simulink model "MOBATSim"  (R2020b)
settings: Solver=FixedStepAuto  StartTime=0.0  StopTime=Sim_t  FixedStep=0.01  MinStep=0.01  RelTol=1e-2
values from neighbouring files (symbols this model uses):
  Vehicles = evalin('base','Vehicles')    [I2V.m]    (also in VehicleSensors.m)
undefined symbols (not defined in the file or in its folder): Sim_Ts
libraries: simulink x50, robotalgslib x10, drivingvehiclecontroller x10, mpcadaslib x10, pid_lib x10
(part 3 of 7)

== system MOBATSim/Vehicle Model 7/Vehicle Model ==
  Longitudinal Speed : Inport
  Steering Angle : Inport  Port=2
  Delay : Delay  DelayLength=1  SampleTime=Sim_Ts
  Kinematic Bicycle Model : Subsystem
  Selector3 : Selector  InputPortWidth=3  IndexOptions=Index vector (dialog)  Indices=[1]  OutputSizes=1
  Selector4 : Selector  InputPortWidth=3  IndexOptions=Index vector (dialog)  Indices=[2]  OutputSizes=1
  Sqrt : Sqrt  SaturateOnIntegerOverflow=on
  Square : Math  Operator=square  SaturateOnIntegerOverflow=on
  Square1 : Math  Operator=square  SaturateOnIntegerOverflow=on
  Sum1 : Sum  Inputs=|++
  Zero-Order Hold1 : ZeroOrderHold  SampleTime=Sim_Ts
  Zero-Order Hold2 : ZeroOrderHold  SampleTime=Sim_Ts
  Pose : Outport
  Speed : Outport  Port=2
  wires:
  Delay/1 -> Speed/1
  Kinematic Bicycle Model/1(state) -> Zero-Order Hold1/1
  Selector4/1 -> Square1/1
  Longitudinal Speed/1 -> Kinematic Bicycle Model/1(v)
  Steering Angle/1 -> Kinematic Bicycle Model/2(Steering Angle)
  Sum1/1 -> Sqrt/1
  Sqrt/1 -> Delay/1
  Square/1 -> Sum1/1
  Square1/1 -> Sum1/2
  Selector3/1 -> Square/1
  Kinematic Bicycle Model/2(stateDot) -> Zero-Order Hold2/1
  Zero-Order Hold1/1 -> Pose/1
  Zero-Order Hold2/1 -> Selector4/1, Selector3/1

== system MOBATSim/Vehicle Model 7/Vehicle Status Check and Acceleration to Speed ==
  note: Longitudinal
  Reference Acceleration : Inport
  Reference Steering Angle : Inport  Port=2
  Acceleration to Speed : Integrator  LimitOutput=on  LowerSaturationLimit=0
  MATLAB System : MATLABSystem  System=VehicleStopStatusCheck  Vehicle_id=Vehicle_id  SimulateUsing=Interpreted execution
      mask Type: VehicleStopStatusCheck
      mask Display:
      | disp('VehicleStopStatusCheck');
      | port_label('input',1,'Acc');
      | port_label('input',2,'Steering');
      | port_label('output',1,'Acc');
      | port_label('output',2,'Stop');
      | port_label('output',3,'Steering');
  Product : Product
  Signal Specification : SignalSpecification  Dimensions=1
  Stop Check : simulink/Logic and Bit Operations/Compare To Constant  relop=~=  const=1  OutDataTypeStr=uint8
  Zero-Order Hold : ZeroOrderHold  SampleTime=Sim_Ts
  Speed Cmd : Outport
  Steering Angle Cmd : Outport  Port=2
  wires:
  Acceleration to Speed/1 -> Signal Specification/1
  Stop Check/1 -> Product/2
  MATLAB System/3 -> Steering Angle Cmd/1
  Signal Specification/1 -> Zero-Order Hold/1
  Reference Acceleration/1 -> MATLAB System/1
  Zero-Order Hold/1 -> Product/1
  Product/1 -> Speed Cmd/1
  MATLAB System/1 -> Acceleration to Speed/1
  Reference Steering Angle/1 -> MATLAB System/2
  MATLAB System/2 -> Stop Check/1

== system MOBATSim/Vehicle Model 8/Longitudinal and Lateral Controllers ==
  Speed Reference : Inport
  Inter Vehicular Distance : Inport  Port=2
  Lead Speed : Inport  Port=3
  drivingMode : Inport  Port=4
  Dist2Stop : Inport  Port=5
  laneChange : Inport  Port=6
  Actual Pose : Inport  Port=7
  Actual Speed : Inport  Port=8
  Lateral Motion Control : Subsystem  Variant=on  VariantControlMode=label  LabelModeActiveChoice=STANLEY  mask{modeLateral=STANLEY}
      mask prompts: modeLateral "Lateral Control Mode:"
      mask TypeOptions modeLateral: PURE_PURSUIT | STANLEY
      mask Callback modeLateral: set_param(gcb,'OverrideUsingVariant',get_param(gcb,'modeLateral'));
  Longitudinal Speed Control : Subsystem
  Longitudinal Acceleration Cmd : Outport
  Reference Steering Angle : Outport  Port=2
  wires:
  laneChange/1 -> Lateral Motion Control/3(changeLane)
  Lateral Motion Control/1(SteerCmd) -> Reference Steering Angle/1
  Actual Speed/1 -> Lateral Motion Control/1(speed), Longitudinal Speed Control/6(Actual Speed)
  drivingMode/1 -> Longitudinal Speed Control/4(Driving Mode)
  Longitudinal Speed Control/1(Longitduinal Acceleration Command) -> Longitudinal Acceleration Cmd/1
  Dist2Stop/1 -> Longitudinal Speed Control/5(Dist2Stop)
  Inter Vehicular Distance/1 -> Longitudinal Speed Control/2(Inter Vehicular Distance)
  Lead Speed/1 -> Longitudinal Speed Control/3(Lead Speed)
  Speed Reference/1 -> Longitudinal Speed Control/1(Speed Reference)
  Actual Pose/1 -> Lateral Motion Control/2(pose)

== system MOBATSim/Vehicle Model 8/Path Planner ==
  note: 1) Add Subsystem or Model blocks as valid variant choices.
      | 2) You cannot connect blocks at this level. At simulation, connectivity is automatically
      | determined, based on the active variant and port name matching.
  CommunicationIDs : Inport
  Astar : Subsystem  VariantControl=Astar
  ShortestPathFinder : Subsystem  VariantControl=ShortestPathFinder
  waypointReached : Outport

== system MOBATSim/Vehicle Model 8/Transform to MOBATSim Coordinates ==
  Pose : Inport
  Constant : Constant  Value=0
  Constant1 : Constant
  Constant2 : Constant  Value=0
  Constant3 : Constant  Value=0
  Constant4 : Constant  Value=pi/2
  Gain : Gain  Gain=-1
  Matrix Concatenate : Concatenate  NumInputs=4  ConcatenateDimension=2
  Matrix Concatenate1 : Concatenate  NumInputs=3  ConcatenateDimension=2
  Selector1 : Selector  InputPortWidth=3  IndexOptions=Index vector (dialog)  Indices=[3]  OutputSizes=1
  Selector3 : Selector  InputPortWidth=3  IndexOptions=Index vector (dialog)  Indices=[1]  OutputSizes=1
  Selector4 : Selector  InputPortWidth=3  IndexOptions=Index vector (dialog)  Indices=[2]  OutputSizes=1
  Sum : Sum  Inputs=|++
  Position : Outport
  Orientation : Outport  Port=2
  wires:
  Sum/1 -> Matrix Concatenate/4
  Constant2/1 -> Matrix Concatenate/1
  Constant3/1 -> Matrix Concatenate1/2
  Gain/1 -> Matrix Concatenate1/3
  Constant4/1 -> Sum/2
  Constant1/1 -> Matrix Concatenate/2
  Selector1/1 -> Sum/1
  Constant/1 -> Matrix Concatenate/3
  Matrix Concatenate/1 -> Orientation/1
  Matrix Concatenate1/1 -> Position/1
  Selector4/1 -> Gain/1
  Selector3/1 -> Matrix Concatenate1/1
  Pose/1 -> Selector1/1, Selector4/1, Selector3/1

== system MOBATSim/Vehicle Model 8/Vehicle Model ==
  Longitudinal Speed : Inport
  Steering Angle : Inport  Port=2
  Delay : Delay  DelayLength=1  SampleTime=Sim_Ts
  Kinematic Bicycle Model : Subsystem
  Selector3 : Selector  InputPortWidth=3  IndexOptions=Index vector (dialog)  Indices=[1]  OutputSizes=1
  Selector4 : Selector  InputPortWidth=3  IndexOptions=Index vector (dialog)  Indices=[2]  OutputSizes=1
  Sqrt : Sqrt  SaturateOnIntegerOverflow=on
  Square : Math  Operator=square  SaturateOnIntegerOverflow=on
  Square1 : Math  Operator=square  SaturateOnIntegerOverflow=on
  Sum1 : Sum  Inputs=|++
  Zero-Order Hold1 : ZeroOrderHold  SampleTime=Sim_Ts
  Zero-Order Hold2 : ZeroOrderHold  SampleTime=Sim_Ts
  Pose : Outport
  Speed : Outport  Port=2
  wires:
  Delay/1 -> Speed/1
  Kinematic Bicycle Model/1(state) -> Zero-Order Hold1/1
  Selector4/1 -> Square1/1
  Longitudinal Speed/1 -> Kinematic Bicycle Model/1(v)
  Steering Angle/1 -> Kinematic Bicycle Model/2(Steering Angle)
  Sum1/1 -> Sqrt/1
  Sqrt/1 -> Delay/1
  Square/1 -> Sum1/1
  Square1/1 -> Sum1/2
  Selector3/1 -> Square/1
  Kinematic Bicycle Model/2(stateDot) -> Zero-Order Hold2/1
  Zero-Order Hold1/1 -> Pose/1
  Zero-Order Hold2/1 -> Selector4/1, Selector3/1

== system MOBATSim/Vehicle Model 8/Vehicle Status Check and Acceleration to Speed ==
  note: Longitudinal
  Reference Acceleration : Inport
  Reference Steering Angle : Inport  Port=2
  Acceleration to Speed : Integrator  LimitOutput=on  LowerSaturationLimit=0
  MATLAB System : MATLABSystem  System=VehicleStopStatusCheck  Vehicle_id=Vehicle_id  SimulateUsing=Interpreted execution
      mask Type: VehicleStopStatusCheck
      mask Display:
      | disp('VehicleStopStatusCheck');
      | port_label('input',1,'Acc');
      | port_label('input',2,'Steering');
      | port_label('output',1,'Acc');
      | port_label('output',2,'Stop');
      | port_label('output',3,'Steering');
  Product : Product
  Signal Specification : SignalSpecification  Dimensions=1
  Stop Check : simulink/Logic and Bit Operations/Compare To Constant  relop=~=  const=1  OutDataTypeStr=uint8
  Zero-Order Hold : ZeroOrderHold  SampleTime=Sim_Ts
  Speed Cmd : Outport
  Steering Angle Cmd : Outport  Port=2
  wires:
  Acceleration to Speed/1 -> Signal Specification/1
  Stop Check/1 -> Product/2
  MATLAB System/3 -> Steering Angle Cmd/1
  Signal Specification/1 -> Zero-Order Hold/1
  Reference Acceleration/1 -> MATLAB System/1
  Zero-Order Hold/1 -> Product/1
  Product/1 -> Speed Cmd/1
  MATLAB System/1 -> Acceleration to Speed/1
  Reference Steering Angle/1 -> MATLAB System/2
  MATLAB System/2 -> Stop Check/1

== system MOBATSim/Vehicle Model 9/Longitudinal and Lateral Controllers ==
  Speed Reference : Inport
  Inter Vehicular Distance : Inport  Port=2
  Lead Speed : Inport  Port=3
  drivingMode : Inport  Port=4
  Dist2Stop : Inport  Port=5
  laneChange : Inport  Port=6
  Actual Pose : Inport  Port=7
  Actual Speed : Inport  Port=8
  Lateral Motion Control : Subsystem  Variant=on  VariantControlMode=label  LabelModeActiveChoice=STANLEY  mask{modeLateral=STANLEY}
      mask prompts: modeLateral "Lateral Control Mode:"
      mask TypeOptions modeLateral: PURE_PURSUIT | STANLEY
      mask Callback modeLateral: set_param(gcb,'OverrideUsingVariant',get_param(gcb,'modeLateral'));
  Longitudinal Speed Control : Subsystem
  Longitudinal Acceleration Cmd : Outport
  Reference Steering Angle : Outport  Port=2
  wires:
  laneChange/1 -> Lateral Motion Control/3(changeLane)
  Lateral Motion Control/1(SteerCmd) -> Reference Steering Angle/1
  Actual Speed/1 -> Lateral Motion Control/1(speed), Longitudinal Speed Control/6(Actual Speed)
  drivingMode/1 -> Longitudinal Speed Control/4(Driving Mode)
  Longitudinal Speed Control/1(Longitduinal Acceleration Command) -> Longitudinal Acceleration Cmd/1
  Dist2Stop/1 -> Longitudinal Speed Control/5(Dist2Stop)
  Inter Vehicular Distance/1 -> Longitudinal Speed Control/2(Inter Vehicular Distance)
  Lead Speed/1 -> Longitudinal Speed Control/3(Lead Speed)
  Speed Reference/1 -> Longitudinal Speed Control/1(Speed Reference)
  Actual Pose/1 -> Lateral Motion Control/2(pose)

== system MOBATSim/Vehicle Model 9/Path Planner ==
  note: 1) Add Subsystem or Model blocks as valid variant choices.
      | 2) You cannot connect blocks at this level. At simulation, connectivity is automatically
      | determined, based on the active variant and port name matching.
  CommunicationIDs : Inport
  Astar : Subsystem  VariantControl=Astar
  ShortestPathFinder : Subsystem  VariantControl=ShortestPathFinder
  waypointReached : Outport

== system MOBATSim/Vehicle Model 9/Transform to MOBATSim Coordinates ==
  Pose : Inport
  Constant : Constant  Value=0
  Constant1 : Constant
  Constant2 : Constant  Value=0
  Constant3 : Constant  Value=0
  Constant4 : Constant  Value=pi/2
  Gain : Gain  Gain=-1
  Matrix Concatenate : Concatenate  NumInputs=4  ConcatenateDimension=2
  Matrix Concatenate1 : Concatenate  NumInputs=3  ConcatenateDimension=2
  Selector1 : Selector  InputPortWidth=3  IndexOptions=Index vector (dialog)  Indices=[3]  OutputSizes=1
  Selector3 : Selector  InputPortWidth=3  IndexOptions=Index vector (dialog)  Indices=[1]  OutputSizes=1
  Selector4 : Selector  InputPortWidth=3  IndexOptions=Index vector (dialog)  Indices=[2]  OutputSizes=1
  Sum : Sum  Inputs=|++
  Position : Outport
  Orientation : Outport  Port=2
  wires:
  Sum/1 -> Matrix Concatenate/4
  Constant2/1 -> Matrix Concatenate/1
  Constant3/1 -> Matrix Concatenate1/2
  Gain/1 -> Matrix Concatenate1/3
  Constant4/1 -> Sum/2
  Constant1/1 -> Matrix Concatenate/2
  Selector1/1 -> Sum/1
  Constant/1 -> Matrix Concatenate/3
  Matrix Concatenate/1 -> Orientation/1
  Matrix Concatenate1/1 -> Position/1
  Selector4/1 -> Gain/1
  Selector3/1 -> Matrix Concatenate1/1
  Pose/1 -> Selector1/1, Selector4/1, Selector3/1

== system MOBATSim/Vehicle Model 9/Vehicle Model ==
  Longitudinal Speed : Inport
  Steering Angle : Inport  Port=2
  Delay : Delay  DelayLength=1  SampleTime=Sim_Ts
  Kinematic Bicycle Model : Subsystem
  Selector3 : Selector  InputPortWidth=3  IndexOptions=Index vector (dialog)  Indices=[1]  OutputSizes=1
  Selector4 : Selector  InputPortWidth=3  IndexOptions=Index vector (dialog)  Indices=[2]  OutputSizes=1
  Sqrt : Sqrt  SaturateOnIntegerOverflow=on
  Square : Math  Operator=square  SaturateOnIntegerOverflow=on
  Square1 : Math  Operator=square  SaturateOnIntegerOverflow=on
  Sum1 : Sum  Inputs=|++
  Zero-Order Hold1 : ZeroOrderHold  SampleTime=Sim_Ts
  Zero-Order Hold2 : ZeroOrderHold  SampleTime=Sim_Ts
  Pose : Outport
  Speed : Outport  Port=2
  wires:
  Delay/1 -> Speed/1
  Kinematic Bicycle Model/1(state) -> Zero-Order Hold1/1
  Selector4/1 -> Square1/1
  Longitudinal Speed/1 -> Kinematic Bicycle Model/1(v)
  Steering Angle/1 -> Kinematic Bicycle Model/2(Steering Angle)
  Sum1/1 -> Sqrt/1
  Sqrt/1 -> Delay/1
  Square/1 -> Sum1/1
  Square1/1 -> Sum1/2
  Selector3/1 -> Square/1
  Kinematic Bicycle Model/2(stateDot) -> Zero-Order Hold2/1
  Zero-Order Hold1/1 -> Pose/1
  Zero-Order Hold2/1 -> Selector4/1, Selector3/1

== system MOBATSim/Vehicle Model 9/Vehicle Status Check and Acceleration to Speed ==
  note: Longitudinal
  Reference Acceleration : Inport
  Reference Steering Angle : Inport  Port=2
  Acceleration to Speed : Integrator  LimitOutput=on  LowerSaturationLimit=0
  MATLAB System : MATLABSystem  System=VehicleStopStatusCheck  Vehicle_id=Vehicle_id  SimulateUsing=Interpreted execution
      mask Type: VehicleStopStatusCheck
      mask Display:
      | disp('VehicleStopStatusCheck');
      | port_label('input',1,'Acc');
      | port_label('input',2,'Steering');
      | port_label('output',1,'Acc');
      | port_label('output',2,'Stop');
      | port_label('output',3,'Steering');
  Product : Product
  Signal Specification : SignalSpecification  Dimensions=1
  Stop Check : simulink/Logic and Bit Operations/Compare To Constant  relop=~=  const=1  OutDataTypeStr=uint8
  Zero-Order Hold : ZeroOrderHold  SampleTime=Sim_Ts
  Speed Cmd : Outport
  Steering Angle Cmd : Outport  Port=2
  wires:
  Acceleration to Speed/1 -> Signal Specification/1
  Stop Check/1 -> Product/2
  MATLAB System/3 -> Steering Angle Cmd/1
  Signal Specification/1 -> Zero-Order Hold/1
  Reference Acceleration/1 -> MATLAB System/1
  Zero-Order Hold/1 -> Product/1
  Product/1 -> Speed Cmd/1
  MATLAB System/1 -> Acceleration to Speed/1
  Reference Steering Angle/1 -> MATLAB System/2
  MATLAB System/2 -> Stop Check/1

== system MOBATSim/Vehicle Model 1/Longitudinal and Lateral Controllers/Lateral Motion Control ==
  note: 1) Add Subsystem or Model blocks as valid variant choices.
      | 2) You cannot connect blocks at this level. At simulation, connectivity is automatically
      | determined, based on the active variant and port name matching.
  speed : Inport
  pose : Inport  Port=2
  changeLane : Inport  Port=3
  Pure Pursuit : Subsystem  VariantControl=PURE_PURSUIT
  Stanley : Subsystem  VariantControl=STANLEY
  SteerCmd : Outport

== system MOBATSim/Vehicle Model 1/Longitudinal and Lateral Controllers/Longitudinal Speed Control ==
  note: The vehicle calculates the speed difference between the actual speed and the reference speed, then generates the acceleration command accordingly.
  Speed Reference : Inport
  Inter Vehicular Distance : Inport  Port=2
  Lead Speed : Inport  Port=3
  Driving Mode : Inport  Port=4
  Dist2Stop : Inport  Port=5
  Actual Speed : Inport  Port=6
  Distance to Stop Controller1 : Subsystem
  Longitudinal Distance Control : Subsystem  Variant=on  VariantControlMode=label  LabelModeActiveChoice=MPC-based  mask{VehicleFollowingControl=MPC-based}
      mask prompts: VehicleFollowingControl "Vehicle Following Control"
      mask TypeOptions VehicleFollowingControl: PID-based | MPC-based
      mask Callback VehicleFollowingControl: set_param(gcb,'OverrideUsingVariant',get_param(gcb,'VehicleFollowingControl'));
      mask Display: image('MOBATSIM-Icon-Set-11 - Platoon.png'); % Use "Edit Image" on toolstrip to change.
  Reference Acceleration Generation : Subsystem
  Reference speed according to the driving mode : Subsystem
  Signal Specification1 : SignalSpecification  Dimensions=1
  Sum13 : Sum  Inputs=|+-
  Longitduinal Acceleration Command : Outport  VectorParamsAs1DForOutWhenUnconnected=off
  wires:
  Longitudinal Distance Control/1(Reference Speed) -> Reference speed according to the driving mode/3(2)
  Lead Speed/1 -> Longitudinal Distance Control/2(Lead Speed)
  Driving Mode/1 -> Reference Acceleration Generation/1(Driving Mode), Reference speed according to the driving mode/1(Driving Mode)
  Signal Specification1/1 -> Longitduinal Acceleration Command/1
  Sum13/1 -> Reference Acceleration Generation/2(Speed Error)
  Inter Vehicular Distance/1 -> Longitudinal Distance Control/1(Relative distance)
  Dist2Stop/1 -> Distance to Stop Controller1/1(Distance to Stop)
  Speed Reference/1 -> Reference speed according to the driving mode/2(1)
  Distance to Stop Controller1/1(ref speed) -> Reference speed according to the driving mode/4(4)
  Reference Acceleration Generation/1(Reference Acceleration Command) -> Signal Specification1/1
  Actual Speed/1 -> Longitudinal Distance Control/3(Ego Speed), Reference Acceleration Generation/3(Actual Speed), Sum13/2
  Reference speed according to the driving mode/1(Reference Speed) -> Sum13/1

== system MOBATSim/Vehicle Model 1/Path Planner/Astar ==
  CommunicationIDs : Inport
  Path Planner - AStar : MATLABSystem  System=VehiclePathPlanner_Astar  Vehicle_id=Vehicle_id  SimulateUsing=Interpreted execution
      mask Type: VehiclePathPlanner_Astar
      mask Display:
      | image('MOBATSIM-Icon-Set_8- Navigation.png');
      | port_label('input',1,'CommunicationIDs');
      | port_label('output',1,'waypointReached');
  waypointReached : Outport
  wires:
  CommunicationIDs/1 -> Path Planner - AStar/1
  Path Planner - AStar/1 -> waypointReached/1

== system MOBATSim/Vehicle Model 1/Path Planner/ShortestPathFinder ==
  CommunicationIDs : Inport
  Path Planner - Shortest : MATLABSystem  System=VehiclePathPlanner_shortestPathFinder  Vehicle_id=Vehicle_id  SimulateUsing=Interpreted execution
      mask Type: VehiclePathPlanner_shortestPathFinder
      mask Display:
      | image('MOBATSIM-Icon-Set_8- Navigation.png');
      | port_label('input',1,'CommunicationIDs');
      | port_label('output',1,'waypointReached');
  waypointReached : Outport
  wires:
  Path Planner - Shortest/1 -> waypointReached/1
  CommunicationIDs/1 -> Path Planner - Shortest/1

== system MOBATSim/Vehicle Model 1/Vehicle Model/Kinematic Bicycle Model ==
  v : Inport
  Steering Angle : Inport  Port=2
  Cos : Trigonometry  Operator=cos
  Gain : Gain  Gain=1/3
  Mux : Mux  Inputs=3
  Mux1 : Mux  Inputs=3
  Product : Product
  Product1 : Product
  Product2 : Product
  Saturation : Saturate  UpperLimit=pi/4  LowerLimit=-pi/4
  Sin : Trigonometry
  Tan : Trigonometry  Operator=tan
  theta : Integrator  InitialCondition=Vehicles(Vehicle_id).dynamics.orientation(4)
  x : Integrator  InitialCondition=Vehicles(Vehicle_id).dynamics.position(1)
  y : Integrator  InitialCondition=-Vehicles(Vehicle_id).dynamics.position(3)
  state : Outport
  stateDot : Outport  Port=2
  wires:
  Tan/1 -> Product2/2
  Product1/1 -> Mux1/2, y/1
  theta/1 -> Cos/1, Sin/1, Mux/3
  v/1 -> Gain/1, Product1/1, Product/1
  Gain/1 -> Product2/1
  Product/1 -> Mux1/1, x/1
  Mux/1 -> state/1
  Sin/1 -> Product1/2
  Steering Angle/1 -> Saturation/1
  Cos/1 -> Product/2
  Product2/1 -> Mux1/3, theta/1
  y/1 -> Mux/2
  x/1 -> Mux/1
  Mux1/1 -> stateDot/1
  Saturation/1 -> Tan/1

== system MOBATSim/Vehicle Model 10/Longitudinal and Lateral Controllers/Lateral Motion Control ==
  note: 1) Add Subsystem or Model blocks as valid variant choices.
      | 2) You cannot connect blocks at this level. At simulation, connectivity is automatically
      | determined, based on the active variant and port name matching.
  speed : Inport
  pose : Inport  Port=2
  changeLane : Inport  Port=3
  Pure Pursuit : Subsystem  VariantControl=PURE_PURSUIT
  Stanley : Subsystem  VariantControl=STANLEY
  SteerCmd : Outport

== system MOBATSim/Vehicle Model 10/Longitudinal and Lateral Controllers/Longitudinal Speed Control ==
  note: The vehicle calculates the speed difference between the actual speed and the reference speed, then generates the acceleration command accordingly.
  Speed Reference : Inport
  Inter Vehicular Distance : Inport  Port=2
  Lead Speed : Inport  Port=3
  Driving Mode : Inport  Port=4
  Dist2Stop : Inport  Port=5
  Actual Speed : Inport  Port=6
  Distance to Stop Controller1 : Subsystem
  Longitudinal Distance Control : Subsystem  Variant=on  VariantControlMode=label  LabelModeActiveChoice=MPC-based  mask{VehicleFollowingControl=MPC-based}
      mask prompts: VehicleFollowingControl "Vehicle Following Control"
      mask TypeOptions VehicleFollowingControl: PID-based | MPC-based
      mask Callback VehicleFollowingControl: set_param(gcb,'OverrideUsingVariant',get_param(gcb,'VehicleFollowingControl'));
      mask Display: image('MOBATSIM-Icon-Set-11 - Platoon.png'); % Use "Edit Image" on toolstrip to change.
  Reference Acceleration Generation : Subsystem
  Reference speed according to the driving mode : Subsystem
  Signal Specification1 : SignalSpecification  Dimensions=1
  Sum13 : Sum  Inputs=|+-
  Longitduinal Acceleration Command : Outport  VectorParamsAs1DForOutWhenUnconnected=off
  wires:
  Longitudinal Distance Control/1(Reference Speed) -> Reference speed according to the driving mode/3(2)
  Lead Speed/1 -> Longitudinal Distance Control/2(Lead Speed)
  Driving Mode/1 -> Reference Acceleration Generation/1(Driving Mode), Reference speed according to the driving mode/1(Driving Mode)
  Signal Specification1/1 -> Longitduinal Acceleration Command/1
  Sum13/1 -> Reference Acceleration Generation/2(Speed Error)
  Inter Vehicular Distance/1 -> Longitudinal Distance Control/1(Relative distance)
  Dist2Stop/1 -> Distance to Stop Controller1/1(Distance to Stop)
  Speed Reference/1 -> Reference speed according to the driving mode/2(1)
  Distance to Stop Controller1/1(ref speed) -> Reference speed according to the driving mode/4(4)
  Reference Acceleration Generation/1(Reference Acceleration Command) -> Signal Specification1/1
  Actual Speed/1 -> Longitudinal Distance Control/3(Ego Speed), Reference Acceleration Generation/3(Actual Speed), Sum13/2
  Reference speed according to the driving mode/1(Reference Speed) -> Sum13/1

== system MOBATSim/Vehicle Model 10/Path Planner/Astar ==
  CommunicationIDs : Inport
  Path Planner - AStar : MATLABSystem  System=VehiclePathPlanner_Astar  Vehicle_id=Vehicle_id  SimulateUsing=Interpreted execution
      mask Type: VehiclePathPlanner_Astar
      mask Display:
      | image('MOBATSIM-Icon-Set_8- Navigation.png');
      | port_label('input',1,'CommunicationIDs');
      | port_label('output',1,'waypointReached');
  waypointReached : Outport
  wires:
  CommunicationIDs/1 -> Path Planner - AStar/1
  Path Planner - AStar/1 -> waypointReached/1

== system MOBATSim/Vehicle Model 10/Path Planner/ShortestPathFinder ==
  CommunicationIDs : Inport
  Path Planner - Shortest : MATLABSystem  System=VehiclePathPlanner_shortestPathFinder  Vehicle_id=Vehicle_id  SimulateUsing=Interpreted execution
      mask Type: VehiclePathPlanner_shortestPathFinder
      mask Display:
      | image('MOBATSIM-Icon-Set_8- Navigation.png');
      | port_label('input',1,'CommunicationIDs');
      | port_label('output',1,'waypointReached');
  waypointReached : Outport
  wires:
  Path Planner - Shortest/1 -> waypointReached/1
  CommunicationIDs/1 -> Path Planner - Shortest/1

== system MOBATSim/Vehicle Model 10/Vehicle Model/Kinematic Bicycle Model ==
  v : Inport
  Steering Angle : Inport  Port=2
  Cos : Trigonometry  Operator=cos
  Gain : Gain  Gain=1/3
  Mux : Mux  Inputs=3
  Mux1 : Mux  Inputs=3
  Product : Product
  Product1 : Product
  Product2 : Product
  Saturation : Saturate  UpperLimit=pi/4  LowerLimit=-pi/4
  Sin : Trigonometry
  Tan : Trigonometry  Operator=tan
  theta : Integrator  InitialCondition=Vehicles(Vehicle_id).dynamics.orientation(4)
  x : Integrator  InitialCondition=Vehicles(Vehicle_id).dynamics.position(1)
  y : Integrator  InitialCondition=-Vehicles(Vehicle_id).dynamics.position(3)
  state : Outport
  stateDot : Outport  Port=2
  wires:
  Tan/1 -> Product2/2
  Product1/1 -> Mux1/2, y/1
  theta/1 -> Cos/1, Sin/1, Mux/3
  v/1 -> Gain/1, Product1/1, Product/1
  Gain/1 -> Product2/1
  Product/1 -> Mux1/1, x/1
  Mux/1 -> state/1
  Sin/1 -> Product1/2
  Steering Angle/1 -> Saturation/1
  Cos/1 -> Product/2
  Product2/1 -> Mux1/3, theta/1
  y/1 -> Mux/2
  x/1 -> Mux/1
  Mux1/1 -> stateDot/1
  Saturation/1 -> Tan/1

== system MOBATSim/Vehicle Model 2/Longitudinal and Lateral Controllers/Lateral Motion Control ==
  note: 1) Add Subsystem or Model blocks as valid variant choices.
      | 2) You cannot connect blocks at this level. At simulation, connectivity is automatically
      | determined, based on the active variant and port name matching.
  speed : Inport
  pose : Inport  Port=2
  changeLane : Inport  Port=3
  Pure Pursuit : Subsystem  VariantControl=PURE_PURSUIT
  Stanley : Subsystem  VariantControl=STANLEY
  SteerCmd : Outport

== system MOBATSim/Vehicle Model 2/Longitudinal and Lateral Controllers/Longitudinal Speed Control ==
  note: The vehicle calculates the speed difference between the actual speed and the reference speed, then generates the acceleration command accordingly.
  Speed Reference : Inport
  Inter Vehicular Distance : Inport  Port=2
  Lead Speed : Inport  Port=3
  Driving Mode : Inport  Port=4
  Dist2Stop : Inport  Port=5
  Actual Speed : Inport  Port=6
  Distance to Stop Controller : Subsystem
  Longitudinal Distance Control : Subsystem  Variant=on  VariantControlMode=label  LabelModeActiveChoice=MPC-based  mask{VehicleFollowingControl=MPC-based}
      mask prompts: VehicleFollowingControl "Vehicle Following Control"
      mask TypeOptions VehicleFollowingControl: PID-based | MPC-based
      mask Callback VehicleFollowingControl: set_param(gcb,'OverrideUsingVariant',get_param(gcb,'VehicleFollowingControl'));
      mask Display: image('MOBATSIM-Icon-Set-11 - Platoon.png'); % Use "Edit Image" on toolstrip to change.
  Reference Acceleration Generation : Subsystem
  Reference speed according to the driving mode : Subsystem
  Signal Specification1 : SignalSpecification  Dimensions=1
  Sum13 : Sum  Inputs=|+-
  Longitduinal Acceleration Command : Outport  VectorParamsAs1DForOutWhenUnconnected=off
  wires:
  Driving Mode/1 -> Reference Acceleration Generation/1(Driving Mode), Reference speed according to the driving mode/1(Driving Mode)
  Signal Specification1/1 -> Longitduinal Acceleration Command/1
  Sum13/1 -> Reference Acceleration Generation/2(Speed Error)
  Dist2Stop/1 -> Distance to Stop Controller/1(Distance to Stop)
  Speed Reference/1 -> Reference speed according to the driving mode/2(1)
  Distance to Stop Controller/1(ref speed) -> Reference speed according to the driving mode/4(4)
  Reference speed according to the driving mode/1(Reference Speed) -> Sum13/1
  Actual Speed/1 -> Longitudinal Distance Control/3(Ego Speed), Reference Acceleration Generation/3(Actual Speed), Sum13/2
  Reference Acceleration Generation/1(Reference Acceleration Command) -> Signal Specification1/1
  Inter Vehicular Distance/1 -> Longitudinal Distance Control/1(Relative distance)
  Lead Speed/1 -> Longitudinal Distance Control/2(Lead Speed)
  Longitudinal Distance Control/1(Reference Speed) -> Reference speed according to the driving mode/3(2)

== system MOBATSim/Vehicle Model 2/Path Planner/Astar ==
  CommunicationIDs : Inport
  Path Planner - AStar : MATLABSystem  System=VehiclePathPlanner_Astar  Vehicle_id=Vehicle_id  SimulateUsing=Interpreted execution
      mask Type: VehiclePathPlanner_Astar
      mask Display:
      | image('MOBATSIM-Icon-Set_8- Navigation.png');
      | port_label('input',1,'CommunicationIDs');
      | port_label('output',1,'waypointReached');
  waypointReached : Outport
  wires:
  CommunicationIDs/1 -> Path Planner - AStar/1
  Path Planner - AStar/1 -> waypointReached/1

== system MOBATSim/Vehicle Model 2/Path Planner/ShortestPathFinder ==
  CommunicationIDs : Inport
  Path Planner - Shortest : MATLABSystem  System=VehiclePathPlanner_shortestPathFinder  Vehicle_id=Vehicle_id  SimulateUsing=Interpreted execution
      mask Type: VehiclePathPlanner_shortestPathFinder
      mask Display:
      | image('MOBATSIM-Icon-Set_8- Navigation.png');
      | port_label('input',1,'CommunicationIDs');
      | port_label('output',1,'waypointReached');
  waypointReached : Outport
  wires:
  Path Planner - Shortest/1 -> waypointReached/1
  CommunicationIDs/1 -> Path Planner - Shortest/1

== system MOBATSim/Vehicle Model 2/Vehicle Model/Kinematic Bicycle Model ==
  v : Inport
  Steering Angle : Inport  Port=2
  Cos : Trigonometry  Operator=cos
  Gain : Gain  Gain=1/3
  Mux : Mux  Inputs=3
  Mux1 : Mux  Inputs=3
  Product : Product
  Product1 : Product
  Product2 : Product
  Saturation : Saturate  UpperLimit=pi/4  LowerLimit=-pi/4
  Sin : Trigonometry
  Tan : Trigonometry  Operator=tan
  theta : Integrator  InitialCondition=Vehicles(Vehicle_id).dynamics.orientation(4)
  x : Integrator  InitialCondition=Vehicles(Vehicle_id).dynamics.position(1)
  y : Integrator  InitialCondition=-Vehicles(Vehicle_id).dynamics.position(3)
  state : Outport
  stateDot : Outport  Port=2
  wires:
  Tan/1 -> Product2/2
  Product1/1 -> Mux1/2, y/1
  theta/1 -> Cos/1, Sin/1, Mux/3
  v/1 -> Gain/1, Product1/1, Product/1
  Gain/1 -> Product2/1
  Product/1 -> Mux1/1, x/1
  Mux/1 -> state/1
  Sin/1 -> Product1/2
  Steering Angle/1 -> Saturation/1
  Cos/1 -> Product/2
  Product2/1 -> Mux1/3, theta/1
  y/1 -> Mux/2
  x/1 -> Mux/1
  Mux1/1 -> stateDot/1
  Saturation/1 -> Tan/1

== system MOBATSim/Vehicle Model 3/Longitudinal and Lateral Controllers/Lateral Motion Control ==
  note: 1) Add Subsystem or Model blocks as valid variant choices.
      | 2) You cannot connect blocks at this level. At simulation, connectivity is automatically
      | determined, based on the active variant and port name matching.
  speed : Inport
  pose : Inport  Port=2
  changeLane : Inport  Port=3
  Pure Pursuit : Subsystem  VariantControl=PURE_PURSUIT
  Stanley : Subsystem  VariantControl=STANLEY
  SteerCmd : Outport

== system MOBATSim/Vehicle Model 3/Longitudinal and Lateral Controllers/Longitudinal Speed Control ==
  note: The vehicle calculates the speed difference between the actual speed and the reference speed, then generates the acceleration command accordingly.
  Speed Reference : Inport
  Inter Vehicular Distance : Inport  Port=2
  Lead Speed : Inport  Port=3
  Driving Mode : Inport  Port=4
  Dist2Stop : Inport  Port=5
  Actual Speed : Inport  Port=6
  Distance to Stop Controller1 : Subsystem
  Longitudinal Distance Control : Subsystem  Variant=on  VariantControlMode=label  LabelModeActiveChoice=MPC-based  mask{VehicleFollowingControl=MPC-based}
      mask prompts: VehicleFollowingControl "Vehicle Following Control"
      mask TypeOptions VehicleFollowingControl: PID-based | MPC-based
      mask Callback VehicleFollowingControl: set_param(gcb,'OverrideUsingVariant',get_param(gcb,'VehicleFollowingControl'));
      mask Display: image('MOBATSIM-Icon-Set-11 - Platoon.png'); % Use "Edit Image" on toolstrip to change.
  Reference Acceleration Generation : Subsystem
  Reference speed according to the driving mode : Subsystem
  Signal Specification1 : SignalSpecification  Dimensions=1
  Sum13 : Sum  Inputs=|+-
  Longitduinal Acceleration Command : Outport  VectorParamsAs1DForOutWhenUnconnected=off
  wires:
  Longitudinal Distance Control/1(Reference Speed) -> Reference speed according to the driving mode/3(2)
  Lead Speed/1 -> Longitudinal Distance Control/2(Lead Speed)
  Driving Mode/1 -> Reference Acceleration Generation/1(Driving Mode), Reference speed according to the driving mode/1(Driving Mode)
  Signal Specification1/1 -> Longitduinal Acceleration Command/1
  Sum13/1 -> Reference Acceleration Generation/2(Speed Error)
  Inter Vehicular Distance/1 -> Longitudinal Distance Control/1(Relative distance)
  Dist2Stop/1 -> Distance to Stop Controller1/1(Distance to Stop)
  Speed Reference/1 -> Reference speed according to the driving mode/2(1)
  Distance to Stop Controller1/1(ref speed) -> Reference speed according to the driving mode/4(4)
  Reference Acceleration Generation/1(Reference Acceleration Command) -> Signal Specification1/1
  Actual Speed/1 -> Longitudinal Distance Control/3(Ego Speed), Reference Acceleration Generation/3(Actual Speed), Sum13/2
  Reference speed according to the driving mode/1(Reference Speed) -> Sum13/1

== system MOBATSim/Vehicle Model 3/Path Planner/Astar ==
  CommunicationIDs : Inport
  Path Planner - AStar : MATLABSystem  System=VehiclePathPlanner_Astar  Vehicle_id=Vehicle_id  SimulateUsing=Interpreted execution
      mask Type: VehiclePathPlanner_Astar
      mask Display:
      | image('MOBATSIM-Icon-Set_8- Navigation.png');
      | port_label('input',1,'CommunicationIDs');
      | port_label('output',1,'waypointReached');
  waypointReached : Outport
  wires:
  CommunicationIDs/1 -> Path Planner - AStar/1
  Path Planner - AStar/1 -> waypointReached/1

== system MOBATSim/Vehicle Model 3/Path Planner/ShortestPathFinder ==
  CommunicationIDs : Inport
  Path Planner - Shortest : MATLABSystem  System=VehiclePathPlanner_shortestPathFinder  Vehicle_id=Vehicle_id  SimulateUsing=Interpreted execution
      mask Type: VehiclePathPlanner_shortestPathFinder
      mask Display:
      | image('MOBATSIM-Icon-Set_8- Navigation.png');
      | port_label('input',1,'CommunicationIDs');
      | port_label('output',1,'waypointReached');
  waypointReached : Outport
  wires:
  Path Planner - Shortest/1 -> waypointReached/1
  CommunicationIDs/1 -> Path Planner - Shortest/1

== system MOBATSim/Vehicle Model 3/Vehicle Model/Kinematic Bicycle Model ==
  v : Inport
  Steering Angle : Inport  Port=2
  Cos : Trigonometry  Operator=cos
  Gain : Gain  Gain=1/3
  Mux : Mux  Inputs=3
  Mux1 : Mux  Inputs=3
  Product : Product
  Product1 : Product
  Product2 : Product
  Saturation : Saturate  UpperLimit=pi/4  LowerLimit=-pi/4
  Sin : Trigonometry
  Tan : Trigonometry  Operator=tan
  theta : Integrator  InitialCondition=Vehicles(Vehicle_id).dynamics.orientation(4)
  x : Integrator  InitialCondition=Vehicles(Vehicle_id).dynamics.position(1)
  y : Integrator  InitialCondition=-Vehicles(Vehicle_id).dynamics.position(3)
  state : Outport
  stateDot : Outport  Port=2
  wires:
  Tan/1 -> Product2/2
  Product1/1 -> Mux1/2, y/1
  theta/1 -> Cos/1, Sin/1, Mux/3
  v/1 -> Gain/1, Product1/1, Product/1
  Gain/1 -> Product2/1
  Product/1 -> Mux1/1, x/1
  Mux/1 -> state/1
  Sin/1 -> Product1/2
  Steering Angle/1 -> Saturation/1
  Cos/1 -> Product/2
  Product2/1 -> Mux1/3, theta/1
  y/1 -> Mux/2
  x/1 -> Mux/1
  Mux1/1 -> stateDot/1
  Saturation/1 -> Tan/1

== system MOBATSim/Vehicle Model 4/Longitudinal and Lateral Controllers/Lateral Motion Control ==
  note: 1) Add Subsystem or Model blocks as valid variant choices.
      | 2) You cannot connect blocks at this level. At simulation, connectivity is automatically
      | determined, based on the active variant and port name matching.
  speed : Inport
  pose : Inport  Port=2
  changeLane : Inport  Port=3
  Pure Pursuit : Subsystem  VariantControl=PURE_PURSUIT
  Stanley : Subsystem  VariantControl=STANLEY
  SteerCmd : Outport

== system MOBATSim/Vehicle Model 4/Longitudinal and Lateral Controllers/Longitudinal Speed Control ==
  note: The vehicle calculates the speed difference between the actual speed and the reference speed, then generates the acceleration command accordingly.
  Speed Reference : Inport
  Inter Vehicular Distance : Inport  Port=2
  Lead Speed : Inport  Port=3
  Driving Mode : Inport  Port=4
  Dist2Stop : Inport  Port=5
  Actual Speed : Inport  Port=6
  Distance to Stop Controller1 : Subsystem
  Longitudinal Distance Control : Subsystem  Variant=on  VariantControlMode=label  LabelModeActiveChoice=MPC-based  mask{VehicleFollowingControl=MPC-based}
      mask prompts: VehicleFollowingControl "Vehicle Following Control"
      mask TypeOptions VehicleFollowingControl: PID-based | MPC-based
      mask Callback VehicleFollowingControl: set_param(gcb,'OverrideUsingVariant',get_param(gcb,'VehicleFollowingControl'));
      mask Display: image('MOBATSIM-Icon-Set-11 - Platoon.png'); % Use "Edit Image" on toolstrip to change.
  Reference Acceleration Generation : Subsystem
  Reference speed according to the driving mode : Subsystem
  Signal Specification1 : SignalSpecification  Dimensions=1
  Sum13 : Sum  Inputs=|+-
  Longitduinal Acceleration Command : Outport  VectorParamsAs1DForOutWhenUnconnected=off
  wires:
  Longitudinal Distance Control/1(Reference Speed) -> Reference speed according to the driving mode/3(2)
  Lead Speed/1 -> Longitudinal Distance Control/2(Lead Speed)
  Driving Mode/1 -> Reference Acceleration Generation/1(Driving Mode), Reference speed according to the driving mode/1(Driving Mode)
  Signal Specification1/1 -> Longitduinal Acceleration Command/1
  Sum13/1 -> Reference Acceleration Generation/2(Speed Error)
  Inter Vehicular Distance/1 -> Longitudinal Distance Control/1(Relative distance)
  Dist2Stop/1 -> Distance to Stop Controller1/1(Distance to Stop)
  Speed Reference/1 -> Reference speed according to the driving mode/2(1)
  Distance to Stop Controller1/1(ref speed) -> Reference speed according to the driving mode/4(4)
  Reference Acceleration Generation/1(Reference Acceleration Command) -> Signal Specification1/1
  Actual Speed/1 -> Longitudinal Distance Control/3(Ego Speed), Reference Acceleration Generation/3(Actual Speed), Sum13/2
  Reference speed according to the driving mode/1(Reference Speed) -> Sum13/1

== system MOBATSim/Vehicle Model 4/Path Planner/Astar ==
  CommunicationIDs : Inport
  Path Planner - AStar : MATLABSystem  System=VehiclePathPlanner_Astar  Vehicle_id=Vehicle_id  SimulateUsing=Interpreted execution
      mask Type: VehiclePathPlanner_Astar
      mask Display:
      | image('MOBATSIM-Icon-Set_8- Navigation.png');
      | port_label('input',1,'CommunicationIDs');
      | port_label('output',1,'waypointReached');
  waypointReached : Outport
  wires:
  CommunicationIDs/1 -> Path Planner - AStar/1
  Path Planner - AStar/1 -> waypointReached/1

== system MOBATSim/Vehicle Model 4/Path Planner/ShortestPathFinder ==
  CommunicationIDs : Inport
  Path Planner - Shortest : MATLABSystem  System=VehiclePathPlanner_shortestPathFinder  Vehicle_id=Vehicle_id  SimulateUsing=Interpreted execution
      mask Type: VehiclePathPlanner_shortestPathFinder
      mask Display:
      | image('MOBATSIM-Icon-Set_8- Navigation.png');
      | port_label('input',1,'CommunicationIDs');
      | port_label('output',1,'waypointReached');
  waypointReached : Outport
  wires:
  Path Planner - Shortest/1 -> waypointReached/1
  CommunicationIDs/1 -> Path Planner - Shortest/1

== system MOBATSim/Vehicle Model 4/Vehicle Model/Kinematic Bicycle Model ==
  v : Inport
  Steering Angle : Inport  Port=2
  Cos : Trigonometry  Operator=cos
  Gain : Gain  Gain=1/3
  Mux : Mux  Inputs=3
  Mux1 : Mux  Inputs=3
  Product : Product
  Product1 : Product
  Product2 : Product
  Saturation : Saturate  UpperLimit=pi/4  LowerLimit=-pi/4
  Sin : Trigonometry
  Tan : Trigonometry  Operator=tan
  theta : Integrator  InitialCondition=Vehicles(Vehicle_id).dynamics.orientation(4)
  x : Integrator  InitialCondition=Vehicles(Vehicle_id).dynamics.position(1)
  y : Integrator  InitialCondition=-Vehicles(Vehicle_id).dynamics.position(3)
  state : Outport
  stateDot : Outport  Port=2
  wires:
  Tan/1 -> Product2/2
  Product1/1 -> Mux1/2, y/1
  theta/1 -> Cos/1, Sin/1, Mux/3
  v/1 -> Gain/1, Product1/1, Product/1
  Gain/1 -> Product2/1
  Product/1 -> Mux1/1, x/1
  Mux/1 -> state/1
  Sin/1 -> Product1/2
  Steering Angle/1 -> Saturation/1
  Cos/1 -> Product/2
  Product2/1 -> Mux1/3, theta/1
  y/1 -> Mux/2
  x/1 -> Mux/1
  Mux1/1 -> stateDot/1
  Saturation/1 -> Tan/1

== system MOBATSim/Vehicle Model 5/Longitudinal and Lateral Controllers/Lateral Motion Control ==
  note: 1) Add Subsystem or Model blocks as valid variant choices.
      | 2) You cannot connect blocks at this level. At simulation, connectivity is automatically
      | determined, based on the active variant and port name matching.
  speed : Inport
  pose : Inport  Port=2
  changeLane : Inport  Port=3
  Pure Pursuit : Subsystem  VariantControl=PURE_PURSUIT
  Stanley : Subsystem  VariantControl=STANLEY
  SteerCmd : Outport

== system MOBATSim/Vehicle Model 5/Longitudinal and Lateral Controllers/Longitudinal Speed Control ==
  note: The vehicle calculates the speed difference between the actual speed and the reference speed, then generates the acceleration command accordingly.
  Speed Reference : Inport
  Inter Vehicular Distance : Inport  Port=2
  Lead Speed : Inport  Port=3
  Driving Mode : Inport  Port=4
  Dist2Stop : Inport  Port=5
  Actual Speed : Inport  Port=6
  Distance to Stop Controller1 : Subsystem
  Longitudinal Distance Control : Subsystem  Variant=on  VariantControlMode=label  LabelModeActiveChoice=MPC-based  mask{VehicleFollowingControl=MPC-based}
      mask prompts: VehicleFollowingControl "Vehicle Following Control"
      mask TypeOptions VehicleFollowingControl: PID-based | MPC-based
      mask Callback VehicleFollowingControl: set_param(gcb,'OverrideUsingVariant',get_param(gcb,'VehicleFollowingControl'));
      mask Display: image('MOBATSIM-Icon-Set-11 - Platoon.png'); % Use "Edit Image" on toolstrip to change.
  Reference Acceleration Generation : Subsystem
  Reference speed according to the driving mode : Subsystem
  Signal Specification1 : SignalSpecification  Dimensions=1
  Sum13 : Sum  Inputs=|+-
  Longitduinal Acceleration Command : Outport  VectorParamsAs1DForOutWhenUnconnected=off
  wires:
  Longitudinal Distance Control/1(Reference Speed) -> Reference speed according to the driving mode/3(2)
  Lead Speed/1 -> Longitudinal Distance Control/2(Lead Speed)
  Driving Mode/1 -> Reference Acceleration Generation/1(Driving Mode), Reference speed according to the driving mode/1(Driving Mode)
  Signal Specification1/1 -> Longitduinal Acceleration Command/1
  Sum13/1 -> Reference Acceleration Generation/2(Speed Error)
  Inter Vehicular Distance/1 -> Longitudinal Distance Control/1(Relative distance)
  Dist2Stop/1 -> Distance to Stop Controller1/1(Distance to Stop)
  Speed Reference/1 -> Reference speed according to the driving mode/2(1)
  Distance to Stop Controller1/1(ref speed) -> Reference speed according to the driving mode/4(4)
  Reference Acceleration Generation/1(Reference Acceleration Command) -> Signal Specification1/1
  Actual Speed/1 -> Longitudinal Distance Control/3(Ego Speed), Reference Acceleration Generation/3(Actual Speed), Sum13/2
  Reference speed according to the driving mode/1(Reference Speed) -> Sum13/1

== system MOBATSim/Vehicle Model 5/Path Planner/Astar ==
  CommunicationIDs : Inport
  Path Planner - AStar : MATLABSystem  System=VehiclePathPlanner_Astar  Vehicle_id=Vehicle_id  SimulateUsing=Interpreted execution
      mask Type: VehiclePathPlanner_Astar
      mask Display:
      | image('MOBATSIM-Icon-Set_8- Navigation.png');
      | port_label('input',1,'CommunicationIDs');
      | port_label('output',1,'waypointReached');
  waypointReached : Outport
  wires:
  CommunicationIDs/1 -> Path Planner - AStar/1
  Path Planner - AStar/1 -> waypointReached/1

== system MOBATSim/Vehicle Model 5/Path Planner/ShortestPathFinder ==
  CommunicationIDs : Inport
  Path Planner - Shortest : MATLABSystem  System=VehiclePathPlanner_shortestPathFinder  Vehicle_id=Vehicle_id  SimulateUsing=Interpreted execution
      mask Type: VehiclePathPlanner_shortestPathFinder
      mask Display:
      | image('MOBATSIM-Icon-Set_8- Navigation.png');
      | port_label('input',1,'CommunicationIDs');
      | port_label('output',1,'waypointReached');
  waypointReached : Outport
  wires:
  Path Planner - Shortest/1 -> waypointReached/1
  CommunicationIDs/1 -> Path Planner - Shortest/1

== system MOBATSim/Vehicle Model 5/Vehicle Model/Kinematic Bicycle Model ==
  v : Inport
  Steering Angle : Inport  Port=2
  Cos : Trigonometry  Operator=cos
  Gain : Gain  Gain=1/3
  Mux : Mux  Inputs=3
  Mux1 : Mux  Inputs=3
  Product : Product
  Product1 : Product
  Product2 : Product
  Saturation : Saturate  UpperLimit=pi/4  LowerLimit=-pi/4
  Sin : Trigonometry
  Tan : Trigonometry  Operator=tan
  theta : Integrator  InitialCondition=Vehicles(Vehicle_id).dynamics.orientation(4)
  x : Integrator  InitialCondition=Vehicles(Vehicle_id).dynamics.position(1)
  y : Integrator  InitialCondition=-Vehicles(Vehicle_id).dynamics.position(3)
  state : Outport
  stateDot : Outport  Port=2
  wires:
  Tan/1 -> Product2/2
  Product1/1 -> Mux1/2, y/1
  theta/1 -> Cos/1, Sin/1, Mux/3
  v/1 -> Gain/1, Product1/1, Product/1
  Gain/1 -> Product2/1
  Product/1 -> Mux1/1, x/1
  Mux/1 -> state/1
  Sin/1 -> Product1/2
  Steering Angle/1 -> Saturation/1
  Cos/1 -> Product/2
  Product2/1 -> Mux1/3, theta/1
  y/1 -> Mux/2
  x/1 -> Mux/1
  Mux1/1 -> stateDot/1
  Saturation/1 -> Tan/1

== system MOBATSim/Vehicle Model 6/Longitudinal and Lateral Controllers/Lateral Motion Control ==
  note: 1) Add Subsystem or Model blocks as valid variant choices.
      | 2) You cannot connect blocks at this level. At simulation, connectivity is automatically
      | determined, based on the active variant and port name matching.
  speed : Inport
  pose : Inport  Port=2
  changeLane : Inport  Port=3
  Pure Pursuit : Subsystem  VariantControl=PURE_PURSUIT
  Stanley : Subsystem  VariantControl=STANLEY
  SteerCmd : Outport

== system MOBATSim/Vehicle Model 6/Longitudinal and Lateral Controllers/Longitudinal Speed Control ==
  note: The vehicle calculates the speed difference between the actual speed and the reference speed, then generates the acceleration command accordingly.
  Speed Reference : Inport
  Inter Vehicular Distance : Inport  Port=2
  Lead Speed : Inport  Port=3
  Driving Mode : Inport  Port=4
  Dist2Stop : Inport  Port=5
  Actual Speed : Inport  Port=6
  Distance to Stop Controller1 : Subsystem
  Longitudinal Distance Control : Subsystem  Variant=on  VariantControlMode=label  LabelModeActiveChoice=MPC-based  mask{VehicleFollowingControl=MPC-based}
      mask prompts: VehicleFollowingControl "Vehicle Following Control"
      mask TypeOptions VehicleFollowingControl: PID-based | MPC-based
      mask Callback VehicleFollowingControl: set_param(gcb,'OverrideUsingVariant',get_param(gcb,'VehicleFollowingControl'));
      mask Display: image('MOBATSIM-Icon-Set-11 - Platoon.png'); % Use "Edit Image" on toolstrip to change.
  Reference Acceleration Generation : Subsystem
  Reference speed according to the driving mode : Subsystem
  Signal Specification1 : SignalSpecification  Dimensions=1
  Sum13 : Sum  Inputs=|+-
  Longitduinal Acceleration Command : Outport  VectorParamsAs1DForOutWhenUnconnected=off
  wires:
  Longitudinal Distance Control/1(Reference Speed) -> Reference speed according to the driving mode/3(2)
  Lead Speed/1 -> Longitudinal Distance Control/2(Lead Speed)
  Driving Mode/1 -> Reference Acceleration Generation/1(Driving Mode), Reference speed according to the driving mode/1(Driving Mode)
  Signal Specification1/1 -> Longitduinal Acceleration Command/1
  Sum13/1 -> Reference Acceleration Generation/2(Speed Error)
  Inter Vehicular Distance/1 -> Longitudinal Distance Control/1(Relative distance)
  Dist2Stop/1 -> Distance to Stop Controller1/1(Distance to Stop)
  Speed Reference/1 -> Reference speed according to the driving mode/2(1)
  Distance to Stop Controller1/1(ref speed) -> Reference speed according to the driving mode/4(4)
  Reference Acceleration Generation/1(Reference Acceleration Command) -> Signal Specification1/1
  Actual Speed/1 -> Longitudinal Distance Control/3(Ego Speed), Reference Acceleration Generation/3(Actual Speed), Sum13/2
  Reference speed according to the driving mode/1(Reference Speed) -> Sum13/1

== system MOBATSim/Vehicle Model 6/Path Planner/Astar ==
  CommunicationIDs : Inport
  Path Planner - AStar : MATLABSystem  System=VehiclePathPlanner_Astar  Vehicle_id=Vehicle_id  SimulateUsing=Interpreted execution
      mask Type: VehiclePathPlanner_Astar
      mask Display:
      | image('MOBATSIM-Icon-Set_8- Navigation.png');
      | port_label('input',1,'CommunicationIDs');
      | port_label('output',1,'waypointReached');
  waypointReached : Outport
  wires:
  CommunicationIDs/1 -> Path Planner - AStar/1
  Path Planner - AStar/1 -> waypointReached/1

== system MOBATSim/Vehicle Model 6/Path Planner/ShortestPathFinder ==
  CommunicationIDs : Inport
  Path Planner - Shortest : MATLABSystem  System=VehiclePathPlanner_shortestPathFinder  Vehicle_id=Vehicle_id  SimulateUsing=Interpreted execution
      mask Type: VehiclePathPlanner_shortestPathFinder
      mask Display:
      | image('MOBATSIM-Icon-Set_8- Navigation.png');
      | port_label('input',1,'CommunicationIDs');
      | port_label('output',1,'waypointReached');
  waypointReached : Outport
  wires:
  Path Planner - Shortest/1 -> waypointReached/1
  CommunicationIDs/1 -> Path Planner - Shortest/1
